simulink library "ConverterPlantLibrary"  (R2026a)
settings: Solver=VariableStepAuto
libraries: nesl_utility x213, fl_lib x211, ee_lib x205
(part 9 of 22)

== system ConverterPlantLibrary/Non-Isolated DC-DC Converters/Non-Isolated DC-DC Converter/NonIsolatedDCDCVariant/SynchronousBoost/MainSwitch/SwitchingMOSFETwithThermal ==
  G : Inport
  MOSFET : ee_lib/Semiconductors & Converters/MOSFET (Ideal, Switching)  PartSpecification="{\"CollectionId\":\"MW.SimscapeElectrical\",\"CollectionVersion\":\"1.0.0\",\"DatasetId\":\"Wolfspeed|C3M0010090K|\",\"DisplayName\":\"Wolfspeed:C3M0010090K\"}"  port_option=ee.enum.controlport.ps  Rds=0.03 % Datasheet derived Ohm  Goff=1e-05 S  Vth=2.4 % Wolfspeed XML derived V  diode_param=ee.enum.semiconductors.protectionDiode.nodynamics  diode_Vf=0.8 V  diode_Ron=1e-3 Ohm  diode_Goff=1e-5 S  diode_C=50e-9 % Parameter not set F  diode_iRM=-235 % Parameter not set A  diode_iF=300 % Parameter not set A  diode_idot=-50 % Parameter not set A/us  diode_trr_param=ee.enum.converters.diodeReverseParam.trr_factor  diode_trr_factor=3 % Parameter not set  diode_trr=15 % Parameter not set us  diode_Qrr=1500 % Parameter not set s*uA  ids_specify=off  ids_priority=None  ids=0 A  ids_nominal_specify=off  ids_nominal_value=1  ids_nominal_unit=A  vds_specify=off  vds_priority=None  vds=0 V  vds_nominal_specify=off  vds_nominal_value=1  vds_nominal_unit=V  vgs_specify=off  vgs_priority=None  vgs=0 V  vgs_nominal_specify=off  vgs_nominal_value=1  vgs_nominal_unit=V  thermal_loss_option=ee.enum.converters.thermalLossOption.tabulated2d  Von_data=[-2.582 -2.511 -2.366 -2.145 -1.916 -1.601 -1.356 -1.103 -0.7517 -0.4733 -0.3149 -0.1528 -0.0851 -0.05 0 0.094 0.161 0.305 0.51 0.83 1.31 1.61 1.908 2.42 2.766 3.142 3.373 3.713;-2.869 -2.757 -2.58 -2.311 -2.042 -1.683 -1.41 -1.134 -0.7615 -0.4747 -0.3153 -0.149 -0.0819 -0.0469 0 0.09975 0.154 0.303 0.509 0.819 1.241 1.581 1.9 2.39 2.758 3.144 3.4 3.78;-4.55 -4.355 -4.055 -3.569 -3.136 -2.526 -2.113 -1.659 -1.117 -0.7115 -0.4389 -0.2087 -0.116 -0.0674 0 0.123 0.239 0.421 0.701 1.175 1.743 2.252 2.7 3.4 4 4.52 5.03 5.4;-5.005 -4.791 -4.461 -3.926 -3.45 -2.779 -2.324 -1.825 -1.229 -0.7826 -0.4828 -0.2296 -0.1276 -0.07414 0 0.1353 0.2629 0.4631 0.7711 1.292 1.917 2.477 2.97 3.74 4.4 4.972 5.533 5.94] % Wolfspeed XML derived V  Tj=[-55 25 150 900] % Wolfspeed XML derived degC  Iout_data=[-311.6 -300 -280 -250 -220 -180 -150 -120 -80 -50 -32.71 -15.83 -9 -5.52 0 9 15.6 30 50 80 120 150 180 220 250 280 300 327] % Wolfspeed XML derived A  tabulateWithVds=true  Eon_data=[0 0.00054 0.00072 0.0009 0.00109 0.00126 0.00142 0.00163 0.0018;0 0.00036 0.00048 0.0006 0.00073 0.00084 0.00095 0.00109 0.0012;0 0.00037 0.00049 0.00061 0.00074 0.00085 0.00097 0.00111 0.00122;0 0.00041 0.00054 0.00067 0.00081 0.00094 0.00106 0.00122 0.00135;0 0.00041 0.00054 0.00067 0.00081 0.00094 0.00106 0.00122 0.00135] % Wolfspeed XML derived J  Eoff_data=[0 0.00013 0.0002 0.00022 0.00026 0.00033 0.00044 0.00055 0.00067;0 0.00014 0.00021 0.00024 0.00028 0.00036 0.00047 0.00059 0.00072;0 0.00016 0.00024 0.00027 0.00031 0.00041 0.00054 0.00067 0.00082;0 0.00016 0.00024 0.00027 0.00032 0.00041 0.00054 0.00068 0.00083;0 0.00016 0.00024 0.00027 0.00032 0.00041 0.00054 0.00068 0.00083] % Wolfspeed XML derived J  Eon_data_3D=reshape([0;0;0;0;0;0;0;0;0;0;0;0;0;0;0;0;0;0;0;0;0;0;0;0;0;0;0;0;0;0;0;0;0;0;0;0;0;0;0;0;0;0;0;0;0;0;0;0;0;0;0;0;0;0;0;0;0;0;0;0;0;0;0;0;0;0;0;0;0;0;0;0;0;0;0;0;0;0;0;0;0;0;0;0;0;0;0;0;0;0;0;0;0;0;0;0.00025;0.00017;0.00017;0.00019;0.00019;0.00035;0.00024;0.00024;0.00026;0.00026;0.00044;0.00029;0.0003;0.00033;0.00033;0.00051;0.00034;0.00035;0.00038;0.00038;0.0006;0.0004;0.00041;0.00045;0.00045;0.00072;0.00048;0.00049;0.00054;0.00054;0.00079;0.00053;0.00054;0.00059;0.00059;0.00087;0.00058;0.00059;0.00065;0.00065;0;0;0;0;0;0.00054;0.00036;0.00037;0.00041;0.00041;0.00072;0.00048;0.00049;0.00054;0.00054;0.0009;0.0006;0.00061;0.00067;0.00067;0.00109;0.00073;0.00074;0.00081;0.00081;0.00126;0.00084;0.00085;0.00094;0.00094;0.00142;0.00095;0.00097;0.00106;0.00106;0.00163;0.00109;0.00111;0.00122;0.00122;0.0018;0.0012;0.00122;0.00135;0.00135],[5 9 4]) % Wolfspeed XML derived J  Eoff_data_3D=reshape([0;0;0;0;0;0;0;0;0;0;0;0;0;0;0;0;0;0;0;0;0;0;0;0;0;0;0;0;0;0;0;0;0;0;0;0;0;0;0;0;0;0;0;0;0;0;0;0;0;0;0;0;0;0;0;0;0;0;0;0;0;0;0;0;0;0;0;0;0;0;0;0;0;0;0;0;0;0;0;0;0;0;0;0;0;0;0;0;0;0;0;0;0;0;0;8e-05;8e-05;0.0001;0.0001;0.0001;0.00014;0.00015;0.00017;0.00017;0.00017;0.00016;0.00018;0.0002;0.0002;0.0002;0.00017;0.00018;0.00021;0.00021;0.00021;0.00023;0.00025;0.00029;0.00029;0.00029;0.0003;0.00032;0.00037;0.00037;0.00037;0.00038;0.00041;0.00046;0.00047;0.00047;0.00046;0.00049;0.00056;0.00057;0.00057;0;0;0;0;0;0.00013;0.00014;0.00016;0.00016;0.00016;0.0002;0.00021;0.00024;0.00024;0.00024;0.00022;0.00024;0.00027;0.00027;0.00027;0.00026;0.00028;0.00031;0.00032;0.00032;0.00033;0.00036;0.00041;0.00041;0.00041;0.00044;0.00047;0.00054;0.00054;0.00054;0.00055;0.00059;0.00067;0.00068;0.00068;0.00067;0.00072;0.00082;0.00083;0.00083],[5 9 4]) % Wolfspeed XML derived J  Tj_loss=[-55 25 150 900 1000] % Wolfspeed XML derived degC  Iout_data_loss=[0 12.2 26.4 38.8 52.6 66 78.9 91 103.3] % Wolfspeed XML derived A  Vds_loss=[-100 0 400 600] % Wolfspeed XML derived V  Eon_scalar=22.86e-3 % Parameter not set J  Eoff_scalar=17.14e-3 % Parameter not set J  Voff=300 % Parameter not set V  Iout_scalar=600 % Parameter not set A  useCurrentFromPreviousCycle=false % Parameter not set  useVoltageFromPreviousCycle=false % Parameter not set  diodeModelType=ee.enum.converters.diodeModelType.pwl  diodeTableType=ee.enum.diode.tableType.VfMat  diode_ReverseIVType=ee.enum.diode.diodeReverseIV.constant  diode_IfMat=[.07, .12, .19, 1.75, 4.24, 7.32, 11.2; .16, .3, .72, 2.14, 4.02, 6.35, 9.12] % Parameter not set A  diode_VfMat=[0 0.718 3.358 3.487 3.935 4.083 4.682 5.031 5.458 5.658 5.958 6.147 6.32 6.575 6.799 7.03 7.267 7.29;0 0.718 2.914 3.116 3.391 3.497 3.954 4.289 4.612 4.933 5.187 5.39 5.581 5.763 6.107 6.422 6.711 6.76;0 0.718 2.4 2.6 2.8 2.982 3.45 3.789 4.099 4.428 4.661 4.85 5.035 5.233 5.51 5.855 6.14 6.19;0 0.6462 2.16 2.34 2.52 2.684 3.105 3.41 3.689 3.985 4.195 4.365 4.532 4.71 4.959 5.269 5.526 5.571;0 0.6462 2.16 2.34 2.52 2.684 3.105 3.41 3.689 3.985 4.195 4.365 4.532 4.71 4.959 5.269 5.526 5.571] % Wolfspeed XML derived V  diode_TjVec=[-55 25 150 900 1000] % Wolfspeed XML derived degC  diode_VfVec=[.5, .7, .9, 1.3, 1.7, 2.1, 2.5] % Parameter not set V  diode_IfVec=[0 0.21 1.74 3.58 8.82 11.74 29.79 49.06 71.98 98.06 121.2 141.4 161.2 181.3 221.3 260.9 300 306.3] % Wolfspeed XML derived A  diode_IrMat=[1e-06, 2e-06, 5e-06, 1e-05, 2.5e-05, 5e-05, .0001; 2e-06, 5e-06, 1e-05, 4e-05, 8e-05, .0002, .0005] % Parameter not set A  diode_VrMat=[10, 100, 200, 250, 300, 325, 350; 10, 70, 160, 220, 270, 300, 320] % Parameter not set V  diode_VrVec=[10, 20, 40, 50, 70, 80, 100] % Parameter not set V  diode_IrVec=[1e-06, 2e-06, 5e-06, 1e-05, 2e-05, 5e-05, .0001] % Parameter not set A  diode_Vr=-600 % Parameter not set V  diode_Ls=150 % Parameter not set nH  diode_Erec=0.03 % Parameter not set J  diode_rec_loss_model=ee.enum.diode.reverseRecoveryModel.fixed  diode_ErecVal=0 % Parameter not set J  diode_scaleWithIandV=false  diode_ErecMat=[0 0;0 0] % Wolfspeed XML derived J  diodeErecMat3D=zeros(2, 3, 2) J  diode_TjrecVec=[25 35] % Wolfspeed XML derived degC  diode_IfrecVec=[0 10] % Wolfspeed XML derived A  diodeVrecVec=[0, 100] V  diode_IrecVal=10 % Parameter not set A  diode_VrecVal=10 % Wolfspeed XML derived V  diode_tFilter=1 / 1000 / 100 % Parameter not set s  separateThermalPortForDiode=false  thermal_network_parameterization=ee.enum.thermalNetworkTopology.external  Rth=[.03, .2] % Parameter not set K/W  Rth_Cauer=[0.01728 0.0646 0.05315 0.1045] % Wolfspeed XML derived K/W  Rth_Foster=[.08, .14, .22, .16] % Parameter not set K/W  thermal_mass_parameterization=ee.enum.thermalNetwork.thermalmass  thermal_mass=[3, 25] % Parameter not set J/K  thermal_mass_Cauer=[0.00466 0.0158 0.0642 0.264] % Wolfspeed XML derived J/K  thermal_mass_Foster=[.001, .005, .05, .5] % Parameter not set J/K  thermal_time_constant=[.1, 5] % Parameter not set s  thermal_time_constant_Cauer=[.1, 1, 5] % Parameter not set s  thermal_time_constant_Foster=[7e-05, .0007, .01, .08] % Parameter not set s  thermal_mass_initial_temperatures=[25, 25] % Parameter not set degC  thermal_mass_initial_temperatures_Cauer=[25 25 25 25] % Wolfspeed XML derived degC  junction_thermal_mass=0.01 % Parameter not set J/K  Tvec_initial_Foster=[25, 25, 25, 25] % Parameter not set degC  RthDiode=[.03, .2] % Parameter not set K/W  RthCauerDiode=[0.01728 0.0646 0.05315 0.1045] % Wolfspeed XML derived K/W  RthFosterDiode=[.03, .2] % Parameter not set K/W  thermalMassDiode=[3, 25] % Parameter not set J/K  thermalMassCauerDiode=[0.00466 0.0158 0.0642 0.264] % Wolfspeed XML derived J/K  thermalMassFosterDiode=[33, 50] % Parameter not set J/K  thermalTauDiode=[.1, 5] % Parameter not set s  thermalTauCauerDiode=[.1, 1, 5] % Parameter not set s  thermalTauFosterDiode=[1, 10] % Parameter not set s  thermalMassInitTempDiode=[25, 25] % Parameter not set degC  thermalMassInitTempCauerDiode=[25 25 25 25] % Wolfspeed XML derived degC  junctionthermalMassDiode=0.1 % Parameter not set J/K  TVecInitialFosterDiode=[25, 25, 25, 25] % Parameter not set degC  no_thermal_network=0 % Parameter not set  mosfet_junction_temperature_specify=on  mosfet_junction_temperature_priority=High  mosfet_junction_temperature=simTemp_K K  mosfet_junction_temperature_nominal_specify=off  mosfet_junction_temperature_nominal_value=1  mosfet_junction_temperature_nominal_unit=degC  diode_junction_temperature_specify=off  diode_junction_temperature_priority=None  diode_junction_temperature=simTemp_K K  diode_junction_temperature_nominal_specify=off  diode_junction_temperature_nominal_value=1  diode_junction_temperature_nominal_unit=degC  Qj_specify=off  Qj_priority=None  Qj=0 W  Qj_nominal_specify=off  Qj_nominal_value=1  Qj_nominal_unit=W  accumulatedSwitchingLosses_specify=off  accumulatedSwitchingLosses_priority=None  accumulatedSwitchingLosses=0 J
      settings: AttributesFormatString=Wolfspeed:C3M0010090K
  SL_PS : nesl_utility/Simulink-PS Converter  PhysicalDomain=network_engine_domain  SubClassName=ps_input  LeftPortType=input  RightPortType=output  PseudoPeriodic=off  Frequencies=[]  NoiseDistribution=none  NoiseParameters=[]  Unit=1  AffineConversion=off  FilteringAndDerivatives=provide  SimscapeFilterOrder=1  InputFilterTimeConstant=0.001  UdotUserProvided=0
  Temperature Source : fl_lib/Thermal/Thermal Sources/Temperature Source  temperature=simTemp_K K
  Thermal Resistor : ee_lib/Passive/Thermal/Thermal Resistor  R=1e-3 K/W  T_specify=off  T_priority=None  T=0 K  T_nominal_specify=off  T_nominal_value=1  T_nominal_unit=K  Q_specify=off  Q_priority=None  Q=0 W  Q_nominal_specify=off  Q_nominal_value=1  Q_nominal_unit=W
  D : PMIOPort  Side=Left
  S : PMIOPort  Port=2  Side=Right
  wires:
  G/1 -> SL_PS/1
  connections:
  Thermal Resistor/RConn1 -- Temperature Source/LConn1
  MOSFET/LConn2 -- Thermal Resistor/LConn1
  MOSFET/RConn2 -- S/RConn1
  MOSFET/RConn1 -- D/RConn1
  SL_PS/RConn1 -- MOSFET/LConn1

== system ConverterPlantLibrary/Non-Isolated DC-DC Converters/Non-Isolated DC-DC Converter/NonIsolatedDCDCVariant/SynchronousBoost/SyncSwitch/IdealSwitch ==
  G : Inport
  SL_PS : nesl_utility/Simulink-PS Converter  PhysicalDomain=network_engine_domain  SubClassName=ps_input  LeftPortType=input  RightPortType=output  PseudoPeriodic=off  Frequencies=[]  NoiseDistribution=none  NoiseParameters=[]  Unit=1  AffineConversion=off  FilteringAndDerivatives=provide  SimscapeFilterOrder=1  InputFilterTimeConstant=0.001  UdotUserProvided=0
  Switch : ee_lib/Semiconductors & Converters/Ideal Semiconductor Switch  port_option=ee.enum.controlport.ps  Ron=RdsOn_SI Ohm  Goff=GdsOff_SI 1/Ohm  Vth=Vth_SI V  diode_param=ee.enum.semiconductors.protectionDiode.nodynamics  diode_Vf=VfBody_SI V  diode_Ron=RdBody_SI Ohm  diode_Goff=GdBody_SI 1/Ohm  diode_C=50e-9 F  diode_iRM=-235 A  diode_iF=300 A  diode_idot=-50 A/us  diode_trr_param=ee.enum.converters.diodetrr.trr_factor  diode_trr_factor=3  diode_trr=15 us  diode_Qrr=1500 s*uA
  D : PMIOPort  Side=Left
  S : PMIOPort  Port=2  Side=Right
  wires:
  G/1 -> SL_PS/1
  connections:
  Switch/RConn2 -- S/RConn1
  Switch/RConn1 -- D/RConn1
  SL_PS/RConn1 -- Switch/LConn1

== system ConverterPlantLibrary/Non-Isolated DC-DC Converters/Non-Isolated DC-DC Converter/NonIsolatedDCDCVariant/SynchronousBoost/SyncSwitch/SwitchingMOSFETwithThermal ==
  G : Inport
  MOSFET : ee_lib/Semiconductors & Converters/MOSFET (Ideal, Switching)  PartSpecification="{\"CollectionId\":\"SimscapeElectrical\",\"CollectionVersion\":\"1.0.0\",\"DatasetId\":\"Wolfspeed|C3M0010090K|\",\"DisplayName\":\"Wolfspeed:C3M0010090K\"}"  port_option=ee.enum.controlport.ps  Rds=0.03 % Datasheet derived Ohm  Goff=1e-05 S  Vth=2.4 % Wolfspeed XML derived V  diode_param=ee.enum.semiconductors.protectionDiode.nodynamics  diode_Vf=0.8 V  diode_Ron=1e-3 Ohm  diode_Goff=1e-5 S  diode_C=50e-9 % Parameter not set F  diode_iRM=-235 % Parameter not set A  diode_iF=300 % Parameter not set A  diode_idot=-50 % Parameter not set A/us  diode_trr_param=ee.enum.converters.diodeReverseParam.trr_factor  diode_trr_factor=3 % Parameter not set  diode_trr=15 % Parameter not set us  diode_Qrr=1500 % Parameter not set s*uA  ids_specify=off  ids_priority=None  ids=0 A  ids_nominal_specify=off  ids_nominal_value=1  ids_nominal_unit=A  vds_specify=off  vds_priority=None  vds=0 V  vds_nominal_specify=off  vds_nominal_value=1  vds_nominal_unit=V  vgs_specify=off  vgs_priority=None  vgs=0 V  vgs_nominal_specify=off  vgs_nominal_value=1  vgs_nominal_unit=V  thermal_loss_option=ee.enum.converters.thermalLossOption.tabulated2d  Von_data=[-2.582 -2.511 -2.366 -2.145 -1.916 -1.601 -1.356 -1.103 -0.7517 -0.4733 -0.3149 -0.1528 -0.0851 -0.05 0 0.094 0.161 0.305 0.51 0.83 1.31 1.61 1.908 2.42 2.766 3.142 3.373 3.713;-2.869 -2.757 -2.58 -2.311 -2.042 -1.683 -1.41 -1.134 -0.7615 -0.4747 -0.3153 -0.149 -0.0819 -0.0469 0 0.09975 0.154 0.303 0.509 0.819 1.241 1.581 1.9 2.39 2.758 3.144 3.4 3.78;-4.55 -4.355 -4.055 -3.569 -3.136 -2.526 -2.113 -1.659 -1.117 -0.7115 -0.4389 -0.2087 -0.116 -0.0674 0 0.123 0.239 0.421 0.701 1.175 1.743 2.252 2.7 3.4 4 4.52 5.03 5.4;-5.005 -4.791 -4.461 -3.926 -3.45 -2.779 -2.324 -1.825 -1.229 -0.7826 -0.4828 -0.2296 -0.1276 -0.07414 0 0.1353 0.2629 0.4631 0.7711 1.292 1.917 2.477 2.97 3.74 4.4 4.972 5.533 5.94] % Wolfspeed XML derived V  Tj=[-55 25 150 900] % Wolfspeed XML derived degC  Iout_data=[-311.6 -300 -280 -250 -220 -180 -150 -120 -80 -50 -32.71 -15.83 -9 -5.52 0 9 15.6 30 50 80 120 150 180 220 250 280 300 327] % Wolfspeed XML derived A  tabulateWithVds=true  Eon_data=[0 0.00054 0.00072 0.0009 0.00109 0.00126 0.00142 0.00163 0.0018;0 0.00036 0.00048 0.0006 0.00073 0.00084 0.00095 0.00109 0.0012;0 0.00037 0.00049 0.00061 0.00074 0.00085 0.00097 0.00111 0.00122;0 0.00041 0.00054 0.00067 0.00081 0.00094 0.00106 0.00122 0.00135;0 0.00041 0.00054 0.00067 0.00081 0.00094 0.00106 0.00122 0.00135] % Wolfspeed XML derived J  Eoff_data=[0 0.00013 0.0002 0.00022 0.00026 0.00033 0.00044 0.00055 0.00067;0 0.00014 0.00021 0.00024 0.00028 0.00036 0.00047 0.00059 0.00072;0 0.00016 0.00024 0.00027 0.00031 0.00041 0.00054 0.00067 0.00082;0 0.00016 0.00024 0.00027 0.00032 0.00041 0.00054 0.00068 0.00083;0 0.00016 0.00024 0.00027 0.00032 0.00041 0.00054 0.00068 0.00083] % Wolfspeed XML derived J  Eon_data_3D=reshape([0;0;0;0;0;0;0;0;0;0;0;0;0;0;0;0;0;0;0;0;0;0;0;0;0;0;0;0;0;0;0;0;0;0;0;0;0;0;0;0;0;0;0;0;0;0;0;0;0;0;0;0;0;0;0;0;0;0;0;0;0;0;0;0;0;0;0;0;0;0;0;0;0;0;0;0;0;0;0;0;0;0;0;0;0;0;0;0;0;0;0;0;0;0;0;0.00025;0.00017;0.00017;0.00019;0.00019;0.00035;0.00024;0.00024;0.00026;0.00026;0.00044;0.00029;0.0003;0.00033;0.00033;0.00051;0.00034;0.00035;0.00038;0.00038;0.0006;0.0004;0.00041;0.00045;0.00045;0.00072;0.00048;0.00049;0.00054;0.00054;0.00079;0.00053;0.00054;0.00059;0.00059;0.00087;0.00058;0.00059;0.00065;0.00065;0;0;0;0;0;0.00054;0.00036;0.00037;0.00041;0.00041;0.00072;0.00048;0.00049;0.00054;0.00054;0.0009;0.0006;0.00061;0.00067;0.00067;0.00109;0.00073;0.00074;0.00081;0.00081;0.00126;0.00084;0.00085;0.00094;0.00094;0.00142;0.00095;0.00097;0.00106;0.00106;0.00163;0.00109;0.00111;0.00122;0.00122;0.0018;0.0012;0.00122;0.00135;0.00135],[5 9 4]) % Wolfspeed XML derived J  Eoff_data_3D=reshape([0;0;0;0;0;0;0;0;0;0;0;0;0;0;0;0;0;0;0;0;0;0;0;0;0;0;0;0;0;0;0;0;0;0;0;0;0;0;0;0;0;0;0;0;0;0;0;0;0;0;0;0;0;0;0;0;0;0;0;0;0;0;0;0;0;0;0;0;0;0;0;0;0;0;0;0;0;0;0;0;0;0;0;0;0;0;0;0;0;0;0;0;0;0;0;8e-05;8e-05;0.0001;0.0001;0.0001;0.00014;0.00015;0.00017;0.00017;0.00017;0.00016;0.00018;0.0002;0.0002;0.0002;0.00017;0.00018;0.00021;0.00021;0.00021;0.00023;0.00025;0.00029;0.00029;0.00029;0.0003;0.00032;0.00037;0.00037;0.00037;0.00038;0.00041;0.00046;0.00047;0.00047;0.00046;0.00049;0.00056;0.00057;0.00057;0;0;0;0;0;0.00013;0.00014;0.00016;0.00016;0.00016;0.0002;0.00021;0.00024;0.00024;0.00024;0.00022;0.00024;0.00027;0.00027;0.00027;0.00026;0.00028;0.00031;0.00032;0.00032;0.00033;0.00036;0.00041;0.00041;0.00041;0.00044;0.00047;0.00054;0.00054;0.00054;0.00055;0.00059;0.00067;0.00068;0.00068;0.00067;0.00072;0.00082;0.00083;0.00083],[5 9 4]) % Wolfspeed XML derived J  Tj_loss=[-55 25 150 900 1000] % Wolfspeed XML derived degC  Iout_data_loss=[0 12.2 26.4 38.8 52.6 66 78.9 91 103.3] % Wolfspeed XML derived A  Vds_loss=[-100 0 400 600] % Wolfspeed XML derived V  Eon_scalar=22.86e-3 % Parameter not set J  Eoff_scalar=17.14e-3 % Parameter not set J  Voff=300 % Parameter not set V  Iout_scalar=600 % Parameter not set A  useCurrentFromPreviousCycle=false % Parameter not set  useVoltageFromPreviousCycle=false % Parameter not set  diodeModelType=ee.enum.converters.diodeModelType.pwl  diodeTableType=ee.enum.diode.tableType.VfMat  diode_ReverseIVType=ee.enum.diode.diodeReverseIV.constant  diode_IfMat=[.07, .12, .19, 1.75, 4.24, 7.32, 11.2; .16, .3, .72, 2.14, 4.02, 6.35, 9.12] % Parameter not set A  diode_VfMat=[0 0.718 3.358 3.487 3.935 4.083 4.682 5.031 5.458 5.658 5.958 6.147 6.32 6.575 6.799 7.03 7.267 7.29;0 0.718 2.914 3.116 3.391 3.497 3.954 4.289 4.612 4.933 5.187 5.39 5.581 5.763 6.107 6.422 6.711 6.76;0 0.718 2.4 2.6 2.8 2.982 3.45 3.789 4.099 4.428 4.661 4.85 5.035 5.233 5.51 5.855 6.14 6.19;0 0.6462 2.16 2.34 2.52 2.684 3.105 3.41 3.689 3.985 4.195 4.365 4.532 4.71 4.959 5.269 5.526 5.571;0 0.6462 2.16 2.34 2.52 2.684 3.105 3.41 3.689 3.985 4.195 4.365 4.532 4.71 4.959 5.269 5.526 5.571] % Wolfspeed XML derived V  diode_TjVec=[-55 25 150 900 1000] % Wolfspeed XML derived degC  diode_VfVec=[.5, .7, .9, 1.3, 1.7, 2.1, 2.5] % Parameter not set V  diode_IfVec=[0 0.21 1.74 3.58 8.82 11.74 29.79 49.06 71.98 98.06 121.2 141.4 161.2 181.3 221.3 260.9 300 306.3] % Wolfspeed XML derived A  diode_IrMat=[1e-06, 2e-06, 5e-06, 1e-05, 2.5e-05, 5e-05, .0001; 2e-06, 5e-06, 1e-05, 4e-05, 8e-05, .0002, .0005] % Parameter not set A  diode_VrMat=[10, 100, 200, 250, 300, 325, 350; 10, 70, 160, 220, 270, 300, 320] % Parameter not set V  diode_VrVec=[10, 20, 40, 50, 70, 80, 100] % Parameter not set V  diode_IrVec=[1e-06, 2e-06, 5e-06, 1e-05, 2e-05, 5e-05, .0001] % Parameter not set A  diode_Vr=-600 % Parameter not set V  diode_Ls=150 % Parameter not set nH  diode_Erec=0.03 % Parameter not set J  diode_rec_loss_model=ee.enum.diode.reverseRecoveryModel.fixed  diode_ErecVal=0 % Parameter not set J  diode_scaleWithIandV=false  diode_ErecMat=[0 0;0 0] % Wolfspeed XML derived J  diodeErecMat3D=zeros(2, 3, 2) J  diode_TjrecVec=[25 35] % Wolfspeed XML derived degC  diode_IfrecVec=[0 10] % Wolfspeed XML derived A  diodeVrecVec=[0, 100] V  diode_IrecVal=10 % Parameter not set A  diode_VrecVal=10 % Wolfspeed XML derived V  diode_tFilter=1 / 1000 / 100 % Parameter not set s  separateThermalPortForDiode=false  thermal_network_parameterization=ee.enum.thermalNetworkTopology.external  Rth=[.03, .2] % Parameter not set K/W  Rth_Cauer=[0.01728 0.0646 0.05315 0.1045] % Wolfspeed XML derived K/W  Rth_Foster=[.08, .14, .22, .16] % Parameter not set K/W  thermal_mass_parameterization=ee.enum.thermalNetwork.thermalmass  thermal_mass=[3, 25] % Parameter not set J/K  thermal_mass_Cauer=[0.00466 0.0158 0.0642 0.264] % Wolfspeed XML derived J/K  thermal_mass_Foster=[.001, .005, .05, .5] % Parameter not set J/K  thermal_time_constant=[.1, 5] % Parameter not set s  thermal_time_constant_Cauer=[.1, 1, 5] % Parameter not set s  thermal_time_constant_Foster=[7e-05, .0007, .01, .08] % Parameter not set s  thermal_mass_initial_temperatures=[25, 25] % Parameter not set degC  thermal_mass_initial_temperatures_Cauer=[25 25 25 25] % Wolfspeed XML derived degC  junction_thermal_mass=0.01 % Parameter not set J/K  Tvec_initial_Foster=[25, 25, 25, 25] % Parameter not set degC  RthDiode=[.03, .2] % Parameter not set K/W  RthCauerDiode=[0.01728 0.0646 0.05315 0.1045] % Wolfspeed XML derived K/W  RthFosterDiode=[.03, .2] % Parameter not set K/W  thermalMassDiode=[3, 25] % Parameter not set J/K  thermalMassCauerDiode=[0.00466 0.0158 0.0642 0.264] % Wolfspeed XML derived J/K  thermalMassFosterDiode=[33, 50] % Parameter not set J/K  thermalTauDiode=[.1, 5] % Parameter not set s  thermalTauCauerDiode=[.1, 1, 5] % Parameter not set s  thermalTauFosterDiode=[1, 10] % Parameter not set s  thermalMassInitTempDiode=[25, 25] % Parameter not set degC  thermalMassInitTempCauerDiode=[25 25 25 25] % Wolfspeed XML derived degC  junctionthermalMassDiode=0.1 % Parameter not set J/K  TVecInitialFosterDiode=[25, 25, 25, 25] % Parameter not set degC  no_thermal_network=0 % Parameter not set  mosfet_junction_temperature_specify=on  mosfet_junction_temperature_priority=High  mosfet_junction_temperature=simTemp_K K  mosfet_junction_temperature_nominal_specify=off  mosfet_junction_temperature_nominal_value=1  mosfet_junction_temperature_nominal_unit=degC  diode_junction_temperature_specify=off  diode_junction_temperature_priority=None  diode_junction_temperature=simTemp_K K  diode_junction_temperature_nominal_specify=off  diode_junction_temperature_nominal_value=1  diode_junction_temperature_nominal_unit=degC  Qj_specify=off  Qj_priority=None  Qj=0 W  Qj_nominal_specify=off  Qj_nominal_value=1  Qj_nominal_unit=W  accumulatedSwitchingLosses_specify=off  accumulatedSwitchingLosses_priority=None  accumulatedSwitchingLosses=0 J
      settings: AttributesFormatString=Wolfspeed:C3M0010090K
  SL_PS : nesl_utility/Simulink-PS Converter  PhysicalDomain=network_engine_domain  SubClassName=ps_input  LeftPortType=input  RightPortType=output  PseudoPeriodic=off  Frequencies=[]  NoiseDistribution=none  NoiseParameters=[]  Unit=1  AffineConversion=off  FilteringAndDerivatives=provide  SimscapeFilterOrder=1  InputFilterTimeConstant=0.001  UdotUserProvided=0
  Temperature Source : fl_lib/Thermal/Thermal Sources/Temperature Source  temperature=simTemp_K K
  Thermal Resistor : ee_lib/Passive/Thermal/Thermal Resistor  R=1e-3 K/W  T_specify=off  T_priority=None  T=0 K  T_nominal_specify=off  T_nominal_value=1  T_nominal_unit=K  Q_specify=off  Q_priority=None  Q=0 W  Q_nominal_specify=off  Q_nominal_value=1  Q_nominal_unit=W
  D : PMIOPort  Side=Left
  S : PMIOPort  Port=2  Side=Right
  wires:
  G/1 -> SL_PS/1
  connections:
  Thermal Resistor/RConn1 -- Temperature Source/LConn1
  MOSFET/LConn2 -- Thermal Resistor/LConn1
  MOSFET/RConn2 -- S/RConn1
  MOSFET/RConn1 -- D/RConn1
  SL_PS/RConn1 -- MOSFET/LConn1

== system ConverterPlantLibrary/Non-Isolated DC-DC Converters/Non-Isolated DC-DC Converter/NonIsolatedDCDCVariant/SynchronousBuck/MainSwitch/IdealSwitch ==
  G : Inport
  SL_PS : nesl_utility/Simulink-PS Converter  PhysicalDomain=network_engine_domain  SubClassName=ps_input  LeftPortType=input  RightPortType=output  PseudoPeriodic=off  Frequencies=[]  NoiseDistribution=none  NoiseParameters=[]  Unit=1  AffineConversion=off  FilteringAndDerivatives=provide  SimscapeFilterOrder=1  InputFilterTimeConstant=0.001  UdotUserProvided=0
  Switch : ee_lib/Semiconductors & Converters/Ideal Semiconductor Switch  port_option=ee.enum.controlport.ps  Ron=RdsOn_SI Ohm  Goff=GdsOff_SI 1/Ohm  Vth=Vth_SI V  diode_param=ee.enum.semiconductors.protectionDiode.nodynamics  diode_Vf=VfBody_SI V  diode_Ron=RdBody_SI Ohm  diode_Goff=GdBody_SI 1/Ohm  diode_C=50e-9 F  diode_iRM=-235 A  diode_iF=300 A  diode_idot=-50 A/us  diode_trr_param=ee.enum.converters.diodetrr.trr_factor  diode_trr_factor=3  diode_trr=15 us  diode_Qrr=1500 s*uA
  D : PMIOPort  Side=Left
  S : PMIOPort  Port=2  Side=Right
  wires:
  G/1 -> SL_PS/1
  connections:
  SL_PS/RConn1 -- Switch/LConn1
  Switch/RConn1 -- D/RConn1
  Switch/RConn2 -- S/RConn1

== system ConverterPlantLibrary/Non-Isolated DC-DC Converters/Non-Isolated DC-DC Converter/NonIsolatedDCDCVariant/SynchronousBuck/MainSwitch/SwitchingMOSFETwithThermal ==
  G : Inport
  MOSFET : ee_lib/Semiconductors & Converters/MOSFET (Ideal, Switching)  PartSpecification="{\"CollectionId\":\"MW.SimscapeElectrical\",\"CollectionVersion\":\"1.0.0\",\"DatasetId\":\"Wolfspeed|C3M0010090K|\",\"DisplayName\":\"Wolfspeed:C3M0010090K\"}"  port_option=ee.enum.controlport.ps  Rds=0.03 % Datasheet derived Ohm  Goff=1e-05 S  Vth=2.41 % Wolfspeed XML derived V  diode_param=ee.enum.semiconductors.protectionDiode.nodynamics  diode_Vf=0.8 V  diode_Ron=1e-3 Ohm  diode_Goff=1e-5 S  diode_C=50e-9 % Parameter not set F  diode_iRM=-235 % Parameter not set A  diode_iF=300 % Parameter not set A  diode_idot=-50 % Parameter not set A/us  diode_trr_param=ee.enum.converters.diodeReverseParam.trr_factor  diode_trr_factor=3 % Parameter not set  diode_trr=15 % Parameter not set us  diode_Qrr=1500 % Parameter not set s*uA  ids_specify=off  ids_priority=None  ids=0 A  ids_nominal_specify=off  ids_nominal_value=1  ids_nominal_unit=A  vds_specify=off  vds_priority=None  vds=0 V  vds_nominal_specify=off  vds_nominal_value=1  vds_nominal_unit=V  vgs_specify=off  vgs_priority=None  vgs=0 V  vgs_nominal_specify=off  vgs_nominal_value=1  vgs_nominal_unit=V  thermal_loss_option=ee.enum.converters.thermalLossOption.tabulated2d  Von_data=[-2.582 -2.511 -2.366 -2.145 -1.916 -1.601 -1.356 -1.103 -0.7517 -0.4733 -0.3149 -0.1528 -0.0851 -0.05 0 0.094 0.161 0.305 0.51 0.83 1.31 1.61 1.908 2.42 2.766 3.142 3.373 3.713;-2.869 -2.757 -2.58 -2.311 -2.042 -1.683 -1.41 -1.134 -0.7615 -0.4747 -0.3153 -0.149 -0.0819 -0.0469 0 0.09975 0.154 0.303 0.509 0.819 1.241 1.581 1.9 2.39 2.758 3.144 3.4 3.78;-4.55 -4.355 -4.055 -3.569 -3.136 -2.526 -2.113 -1.659 -1.117 -0.7115 -0.4389 -0.2087 -0.116 -0.0674 0 0.123 0.239 0.421 0.701 1.175 1.743 2.252 2.7 3.4 4 4.52 5.03 5.4;-5.005 -4.791 -4.461 -3.926 -3.45 -2.779 -2.324 -1.825 -1.229 -0.7826 -0.4828 -0.2296 -0.1276 -0.07414 0 0.1353 0.2629 0.4631 0.7711 1.292 1.917 2.477 2.97 3.74 4.4 4.972 5.533 5.94] % Wolfspeed XML derived V  Tj=[-55 25 150 900] % Wolfspeed XML derived degC  Iout_data=[-311.6 -300 -280 -250 -220 -180 -150 -120 -80 -50 -32.71 -15.83 -9 -5.52 0 9 15.6 30 50 80 120 150 180 220 250 280 300 327] % Wolfspeed XML derived A  tabulateWithVds=true  Eon_data=[0 0.00054 0.00072 0.0009 0.00109 0.00126 0.00142 0.00163 0.0018;0 0.00036 0.00048 0.0006 0.00073 0.00084 0.00095 0.00109 0.0012;0 0.00037 0.00049 0.00061 0.00074 0.00085 0.00097 0.00111 0.00122;0 0.00041 0.00054 0.00067 0.00081 0.00094 0.00106 0.00122 0.00135;0 0.00041 0.00054 0.00067 0.00081 0.00094 0.00106 0.00122 0.00135] % Wolfspeed XML derived J  Eoff_data=[0 0.00013 0.0002 0.00022 0.00026 0.00033 0.00044 0.00055 0.00067;0 0.00014 0.00021 0.00024 0.00028 0.00036 0.00047 0.00059 0.00072;0 0.00016 0.00024 0.00027 0.00031 0.00041 0.00054 0.00067 0.00082;0 0.00016 0.00024 0.00027 0.00032 0.00041 0.00054 0.00068 0.00083;0 0.00016 0.00024 0.00027 0.00032 0.00041 0.00054 0.00068 0.00083] % Wolfspeed XML derived J  Eon_data_3D=reshape([0;0;0;0;0;0;0;0;0;0;0;0;0;0;0;0;0;0;0;0;0;0;0;0;0;0;0;0;0;0;0;0;0;0;0;0;0;0;0;0;0;0;0;0;0;0;0;0;0;0;0;0;0;0;0;0;0;0;0;0;0;0;0;0;0;0;0;0;0;0;0;0;0;0;0;0;0;0;0;0;0;0;0;0;0;0;0;0;0;0;0;0;0;0;0;0.00025;0.00017;0.00017;0.00019;0.00019;0.00035;0.00024;0.00024;0.00026;0.00026;0.00044;0.00029;0.0003;0.00033;0.00033;0.00051;0.00034;0.00035;0.00038;0.00038;0.0006;0.0004;0.00041;0.00045;0.00045;0.00072;0.00048;0.00049;0.00054;0.00054;0.00079;0.00053;0.00054;0.00059;0.00059;0.00087;0.00058;0.00059;0.00065;0.00065;0;0;0;0;0;0.00054;0.00036;0.00037;0.00041;0.00041;0.00072;0.00048;0.00049;0.00054;0.00054;0.0009;0.0006;0.00061;0.00067;0.00067;0.00109;0.00073;0.00074;0.00081;0.00081;0.00126;0.00084;0.00085;0.00094;0.00094;0.00142;0.00095;0.00097;0.00106;0.00106;0.00163;0.00109;0.00111;0.00122;0.00122;0.0018;0.0012;0.00122;0.00135;0.00135],[5 9 4]) % Wolfspeed XML derived J  Eoff_data_3D=reshape([0;0;0;0;0;0;0;0;0;0;0;0;0;0;0;0;0;0;0;0;0;0;0;0;0;0;0;0;0;0;0;0;0;0;0;0;0;0;0;0;0;0;0;0;0;0;0;0;0;0;0;0;0;0;0;0;0;0;0;0;0;0;0;0;0;0;0;0;0;0;0;0;0;0;0;0;0;0;0;0;0;0;0;0;0;0;0;0;0;0;0;0;0;0;0;8e-05;8e-05;0.0001;0.0001;0.0001;0.00014;0.00015;0.00017;0.00017;0.00017;0.00016;0.00018;0.0002;0.0002;0.0002;0.00017;0.00018;0.00021;0.00021;0.00021;0.00023;0.00025;0.00029;0.00029;0.00029;0.0003;0.00032;0.00037;0.00037;0.00037;0.00038;0.00041;0.00046;0.00047;0.00047;0.00046;0.00049;0.00056;0.00057;0.00057;0;0;0;0;0;0.00013;0.00014;0.00016;0.00016;0.00016;0.0002;0.00021;0.00024;0.00024;0.00024;0.00022;0.00024;0.00027;0.00027;0.00027;0.00026;0.00028;0.00031;0.00032;0.00032;0.00033;0.00036;0.00041;0.00041;0.00041;0.00044;0.00047;0.00054;0.00054;0.00054;0.00055;0.00059;0.00067;0.00068;0.00068;0.00067;0.00072;0.00082;0.00083;0.00083],[5 9 4]) % Wolfspeed XML derived J  Tj_loss=[-55 25 150 900 1000] % Wolfspeed XML derived degC  Iout_data_loss=[0 12.2 26.4 38.8 52.6 66 78.9 91 103.3] % Wolfspeed XML derived A  Vds_loss=[-100 0 400 600] % Wolfspeed XML derived V  Eon_scalar=22.86e-3 % Parameter not set J  Eoff_scalar=17.14e-3 % Parameter not set J  Voff=300 % Parameter not set V  Iout_scalar=600 % Parameter not set A  useCurrentFromPreviousCycle=false % Parameter not set  useVoltageFromPreviousCycle=false % Parameter not set  diodeModelType=ee.enum.converters.diodeModelType.pwl  diodeTableType=ee.enum.diode.tableType.VfMat  diode_ReverseIVType=ee.enum.diode.diodeReverseIV.constant  diode_IfMat=[.07, .12, .19, 1.75, 4.24, 7.32, 11.2; .16, .3, .72, 2.14, 4.02, 6.35, 9.12] % Parameter not set A  diode_VfMat=[0 0.718 3.358 3.487 3.935 4.083 4.682 5.031 5.458 5.658 5.958 6.147 6.32 6.575 6.799 7.03 7.267 7.29;0 0.718 2.914 3.116 3.391 3.497 3.954 4.289 4.612 4.933 5.187 5.39 5.581 5.763 6.107 6.422 6.711 6.76;0 0.718 2.4 2.6 2.8 2.982 3.45 3.789 4.099 4.428 4.661 4.85 5.035 5.233 5.51 5.855 6.14 6.19;0 0.6462 2.16 2.34 2.52 2.684 3.105 3.41 3.689 3.985 4.195 4.365 4.532 4.71 4.959 5.269 5.526 5.571;0 0.6462 2.16 2.34 2.52 2.684 3.105 3.41 3.689 3.985 4.195 4.365 4.532 4.71 4.959 5.269 5.526 5.571] % Wolfspeed XML derived V  diode_TjVec=[-55 25 150 900 1000] % Wolfspeed XML derived degC  diode_VfVec=[.5, .7, .9, 1.3, 1.7, 2.1, 2.5] % Parameter not set V  diode_IfVec=[0 0.21 1.74 3.58 8.82 11.74 29.79 49.06 71.98 98.06 121.2 141.4 161.2 181.3 221.3 260.9 300 306.3] % Wolfspeed XML derived A  diode_IrMat=[1e-06, 2e-06, 5e-06, 1e-05, 2.5e-05, 5e-05, .0001; 2e-06, 5e-06, 1e-05, 4e-05, 8e-05, .0002, .0005] % Parameter not set A  diode_VrMat=[10, 100, 200, 250, 300, 325, 350; 10, 70, 160, 220, 270, 300, 320] % Parameter not set V  diode_VrVec=[10, 20, 40, 50, 70, 80, 100] % Parameter not set V  diode_IrVec=[1e-06, 2e-06, 5e-06, 1e-05, 2e-05, 5e-05, .0001] % Parameter not set A  diode_Vr=-600 % Parameter not set V  diode_Ls=150 % Parameter not set nH  diode_Erec=0.03 % Parameter not set J  diode_rec_loss_model=ee.enum.diode.reverseRecoveryModel.fixed  diode_ErecVal=0 % Parameter not set J  diode_scaleWithIandV=false  diode_ErecMat=[0 0;0 0] % Wolfspeed XML derived J  diodeErecMat3D=zeros(2, 3, 2) J  diode_TjrecVec=[25 35] % Wolfspeed XML derived degC  diode_IfrecVec=[0 10] % Wolfspeed XML derived A  diodeVrecVec=[0, 100] V  diode_IrecVal=10 % Parameter not set A  diode_VrecVal=10 % Wolfspeed XML derived V  diode_tFilter=1 / 1000 / 100 % Parameter not set s  separateThermalPortForDiode=false  thermal_network_parameterization=ee.enum.thermalNetworkTopology.external  Rth=[.03, .2] % Parameter not set K/W  Rth_Cauer=[0.01728 0.0646 0.05315 0.1045] % Wolfspeed XML derived K/W  Rth_Foster=[.08, .14, .22, .16] % Parameter not set K/W  thermal_mass_parameterization=ee.enum.thermalNetwork.thermalmass  thermal_mass=[3, 25] % Parameter not set J/K  thermal_mass_Cauer=[0.00466 0.0158 0.0642 0.264] % Wolfspeed XML derived J/K  thermal_mass_Foster=[.001, .005, .05, .5] % Parameter not set J/K  thermal_time_constant=[.1, 5] % Parameter not set s  thermal_time_constant_Cauer=[.1, 1, 5] % Parameter not set s  thermal_time_constant_Foster=[7e-05, .0007, .01, .08] % Parameter not set s  thermal_mass_initial_temperatures=[25, 25] % Parameter not set degC  thermal_mass_initial_temperatures_Cauer=[25 25 25 25] % Wolfspeed XML derived degC  junction_thermal_mass=0.01 % Parameter not set J/K  Tvec_initial_Foster=[25, 25, 25, 25] % Parameter not set degC  RthDiode=[.03, .2] % Parameter not set K/W  RthCauerDiode=[0.01728 0.0646 0.05315 0.1045] % Wolfspeed XML derived K/W  RthFosterDiode=[.03, .2] % Parameter not set K/W  thermalMassDiode=[3, 25] % Parameter not set J/K  thermalMassCauerDiode=[0.00466 0.0158 0.0642 0.264] % Wolfspeed XML derived J/K  thermalMassFosterDiode=[33, 50] % Parameter not set J/K  thermalTauDiode=[.1, 5] % Parameter not set s  thermalTauCauerDiode=[.1, 1, 5] % Parameter not set s  thermalTauFosterDiode=[1, 10] % Parameter not set s  thermalMassInitTempDiode=[25, 25] % Parameter not set degC  thermalMassInitTempCauerDiode=[25 25 25 25] % Wolfspeed XML derived degC  junctionthermalMassDiode=0.1 % Parameter not set J/K  TVecInitialFosterDiode=[25, 25, 25, 25] % Parameter not set degC  no_thermal_network=0 % Parameter not set  mosfet_junction_temperature_specify=on  mosfet_junction_temperature_priority=High  mosfet_junction_temperature=simTemp_K K  mosfet_junction_temperature_nominal_specify=off  mosfet_junction_temperature_nominal_value=1  mosfet_junction_temperature_nominal_unit=degC  diode_junction_temperature_specify=off  diode_junction_temperature_priority=None  diode_junction_temperature=simTemp_K K  diode_junction_temperature_nominal_specify=off  diode_junction_temperature_nominal_value=1  diode_junction_temperature_nominal_unit=degC  Qj_specify=off  Qj_priority=None  Qj=0 W  Qj_nominal_specify=off  Qj_nominal_value=1  Qj_nominal_unit=W  accumulatedSwitchingLosses_specify=off  accumulatedSwitchingLosses_priority=None  accumulatedSwitchingLosses=0 J
      settings: AttributesFormatString=Wolfspeed:C3M0010090K
  SL_PS : nesl_utility/Simulink-PS Converter  PhysicalDomain=network_engine_domain  SubClassName=ps_input  LeftPortType=input  RightPortType=output  PseudoPeriodic=off  Frequencies=[]  NoiseDistribution=none  NoiseParameters=[]  Unit=1  AffineConversion=off  FilteringAndDerivatives=provide  SimscapeFilterOrder=1  InputFilterTimeConstant=0.001  UdotUserProvided=0
  Temperature Source : fl_lib/Thermal/Thermal Sources/Temperature Source  temperature=simTemp_K K
  Thermal Resistor : ee_lib/Passive/Thermal/Thermal Resistor  R=1e-3 K/W  T_specify=off  T_priority=None  T=0 K  T_nominal_specify=off  T_nominal_value=1  T_nominal_unit=K  Q_specify=off  Q_priority=None  Q=0 W  Q_nominal_specify=off  Q_nominal_value=1  Q_nominal_unit=W
  D : PMIOPort  Side=Left
  S : PMIOPort  Port=2  Side=Right
  wires:
  G/1 -> SL_PS/1
  connections:
  SL_PS/RConn1 -- MOSFET/LConn1
  MOSFET/RConn1 -- D/RConn1
  MOSFET/RConn2 -- S/RConn1
  MOSFET/LConn2 -- Thermal Resistor/LConn1
  Thermal Resistor/RConn1 -- Temperature Source/LConn1

== system ConverterPlantLibrary/Non-Isolated DC-DC Converters/Non-Isolated DC-DC Converter/NonIsolatedDCDCVariant/SynchronousBuck/SyncSwitch/IdealSwitch ==
  G : Inport
  SL_PS : nesl_utility/Simulink-PS Converter  PhysicalDomain=network_engine_domain  SubClassName=ps_input  LeftPortType=input  RightPortType=output  PseudoPeriodic=off  Frequencies=[]  NoiseDistribution=none  NoiseParameters=[]  Unit=1  AffineConversion=off  FilteringAndDerivatives=provide  SimscapeFilterOrder=1  InputFilterTimeConstant=0.001  UdotUserProvided=0
  Switch : ee_lib/Semiconductors & Converters/Ideal Semiconductor Switch  port_option=ee.enum.controlport.ps  Ron=RdsOn_SI Ohm  Goff=GdsOff_SI 1/Ohm  Vth=Vth_SI V  diode_param=ee.enum.semiconductors.protectionDiode.nodynamics  diode_Vf=VfBody_SI V  diode_Ron=RdBody_SI Ohm  diode_Goff=GdBody_SI 1/Ohm  diode_C=50e-9 F  diode_iRM=-235 A  diode_iF=300 A  diode_idot=-50 A/us  diode_trr_param=ee.enum.converters.diodetrr.trr_factor  diode_trr_factor=3  diode_trr=15 us  diode_Qrr=1500 s*uA
  D : PMIOPort  Side=Left
  S : PMIOPort  Port=2  Side=Right
  wires:
  G/1 -> SL_PS/1
  connections:
  SL_PS/RConn1 -- Switch/LConn1
  Switch/RConn1 -- D/RConn1
  Switch/RConn2 -- S/RConn1

== system ConverterPlantLibrary/Non-Isolated DC-DC Converters/Non-Isolated DC-DC Converter/NonIsolatedDCDCVariant/SynchronousBuck/SyncSwitch/SwitchingMOSFETwithThermal ==
  G : Inport
  MOSFET : ee_lib/Semiconductors & Converters/MOSFET (Ideal, Switching)  PartSpecification="{\"CollectionId\":\"SimscapeElectrical\",\"CollectionVersion\":\"1.0.0\",\"DatasetId\":\"Wolfspeed|C3M0010090K|\",\"DisplayName\":\"Wolfspeed:C3M0010090K\"}"  port_option=ee.enum.controlport.ps  Rds=0.03 % Datasheet derived Ohm  Goff=1e-05 S  Vth=2.41 % Wolfspeed XML derived V  diode_param=ee.enum.semiconductors.protectionDiode.nodynamics  diode_Vf=0.8 V  diode_Ron=1e-3 Ohm  diode_Goff=1e-5 S  diode_C=50e-9 % Parameter not set F  diode_iRM=-235 % Parameter not set A  diode_iF=300 % Parameter not set A  diode_idot=-50 % Parameter not set A/us  diode_trr_param=ee.enum.converters.diodeReverseParam.trr_factor  diode_trr_factor=3 % Parameter not set  diode_trr=15 % Parameter not set us  diode_Qrr=1500 % Parameter not set s*uA  ids_specify=off  ids_priority=None  ids=0 A  ids_nominal_specify=off  ids_nominal_value=1  ids_nominal_unit=A  vds_specify=off  vds_priority=None  vds=0 V  vds_nominal_specify=off  vds_nominal_value=1  vds_nominal_unit=V  vgs_specify=off  vgs_priority=None  vgs=0 V  vgs_nominal_specify=off  vgs_nominal_value=1  vgs_nominal_unit=V  thermal_loss_option=ee.enum.converters.thermalLossOption.tabulated2d  Von_data=[-2.582 -2.511 -2.366 -2.145 -1.916 -1.601 -1.356 -1.103 -0.7517 -0.4733 -0.3149 -0.1528 -0.0851 -0.05 0 0.094 0.161 0.305 0.51 0.83 1.31 1.61 1.908 2.42 2.766 3.142 3.373 3.713;-2.869 -2.757 -2.58 -2.311 -2.042 -1.683 -1.41 -1.134 -0.7615 -0.4747 -0.3153 -0.149 -0.0819 -0.0469 0 0.09975 0.154 0.303 0.509 0.819 1.241 1.581 1.9 2.39 2.758 3.144 3.4 3.78;-4.55 -4.355 -4.055 -3.569 -3.136 -2.526 -2.113 -1.659 -1.117 -0.7115 -0.4389 -0.2087 -0.116 -0.0674 0 0.123 0.239 0.421 0.701 1.175 1.743 2.252 2.7 3.4 4 4.52 5.03 5.4;-5.005 -4.791 -4.461 -3.926 -3.45 -2.779 -2.324 -1.825 -1.229 -0.7826 -0.4828 -0.2296 -0.1276 -0.07414 0 0.1353 0.2629 0.4631 0.7711 1.292 1.917 2.477 2.97 3.74 4.4 4.972 5.533 5.94] % Wolfspeed XML derived V  Tj=[-55 25 150 900] % Wolfspeed XML derived degC  Iout_data=[-311.6 -300 -280 -250 -220 -180 -150 -120 -80 -50 -32.71 -15.83 -9 -5.52 0 9 15.6 30 50 80 120 150 180 220 250 280 300 327] % Wolfspeed XML derived A  tabulateWithVds=true  Eon_data=[0 0.00054 0.00072 0.0009 0.00109 0.00126 0.00142 0.00163 0.0018;0 0.00036 0.00048 0.0006 0.00073 0.00084 0.00095 0.00109 0.0012;0 0.00037 0.00049 0.00061 0.00074 0.00085 0.00097 0.00111 0.00122;0 0.00041 0.00054 0.00067 0.00081 0.00094 0.00106 0.00122 0.00135;0 0.00041 0.00054 0.00067 0.00081 0.00094 0.00106 0.00122 0.00135] % Wolfspeed XML derived J  Eoff_data=[0 0.00013 0.0002 0.00022 0.00026 0.00033 0.00044 0.00055 0.00067;0 0.00014 0.00021 0.00024 0.00028 0.00036 0.00047 0.00059 0.00072;0 0.00016 0.00024 0.00027 0.00031 0.00041 0.00054 0.00067 0.00082;0 0.00016 0.00024 0.00027 0.00032 0.00041 0.00054 0.00068 0.00083;0 0.00016 0.00024 0.00027 0.00032 0.00041 0.00054 0.00068 0.00083] % Wolfspeed XML derived J  Eon_data_3D=reshape([0;0;0;0;0;0;0;0;0;0;0;0;0;0;0;0;0;0;0;0;0;0;0;0;0;0;0;0;0;0;0;0;0;0;0;0;0;0;0;0;0;0;0;0;0;0;0;0;0;0;0;0;0;0;0;0;0;0;0;0;0;0;0;0;0;0;0;0;0;0;0;0;0;0;0;0;0;0;0;0;0;0;0;0;0;0;0;0;0;0;0;0;0;0;0;0.00025;0.00017;0.00017;0.00019;0.00019;0.00035;0.00024;0.00024;0.00026;0.00026;0.00044;0.00029;0.0003;0.00033;0.00033;0.00051;0.00034;0.00035;0.00038;0.00038;0.0006;0.0004;0.00041;0.00045;0.00045;0.00072;0.00048;0.00049;0.00054;0.00054;0.00079;0.00053;0.00054;0.00059;0.00059;0.00087;0.00058;0.00059;0.00065;0.00065;0;0;0;0;0;0.00054;0.00036;0.00037;0.00041;0.00041;0.00072;0.00048;0.00049;0.00054;0.00054;0.0009;0.0006;0.00061;0.00067;0.00067;0.00109;0.00073;0.00074;0.00081;0.00081;0.00126;0.00084;0.00085;0.00094;0.00094;0.00142;0.00095;0.00097;0.00106;0.00106;0.00163;0.00109;0.00111;0.00122;0.00122;0.0018;0.0012;0.00122;0.00135;0.00135],[5 9 4]) % Wolfspeed XML derived J  Eoff_data_3D=reshape([0;0;0;0;0;0;0;0;0;0;0;0;0;0;0;0;0;0;0;0;0;0;0;0;0;0;0;0;0;0;0;0;0;0;0;0;0;0;0;0;0;0;0;0;0;0;0;0;0;0;0;0;0;0;0;0;0;0;0;0;0;0;0;0;0;0;0;0;0;0;0;0;0;0;0;0;0;0;0;0;0;0;0;0;0;0;0;0;0;0;0;0;0;0;0;8e-05;8e-05;0.0001;0.0001;0.0001;0.00014;0.00015;0.00017;0.00017;0.00017;0.00016;0.00018;0.0002;0.0002;0.0002;0.00017;0.00018;0.00021;0.00021;0.00021;0.00023;0.00025;0.00029;0.00029;0.00029;0.0003;0.00032;0.00037;0.00037;0.00037;0.00038;0.00041;0.00046;0.00047;0.00047;0.00046;0.00049;0.00056;0.00057;0.00057;0;0;0;0;0;0.00013;0.00014;0.00016;0.00016;0.00016;0.0002;0.00021;0.00024;0.00024;0.00024;0.00022;0.00024;0.00027;0.00027;0.00027;0.00026;0.00028;0.00031;0.00032;0.00032;0.00033;0.00036;0.00041;0.00041;0.00041;0.00044;0.00047;0.00054;0.00054;0.00054;0.00055;0.00059;0.00067;0.00068;0.00068;0.00067;0.00072;0.00082;0.00083;0.00083],[5 9 4]) % Wolfspeed XML derived J  Tj_loss=[-55 25 150 900 1000] % Wolfspeed XML derived degC  Iout_data_loss=[0 12.2 26.4 38.8 52.6 66 78.9 91 103.3] % Wolfspeed XML derived A  Vds_loss=[-100 0 400 600] % Wolfspeed XML derived V  Eon_scalar=22.86e-3 % Parameter not set J  Eoff_scalar=17.14e-3 % Parameter not set J  Voff=300 % Parameter not set V  Iout_scalar=600 % Parameter not set A  useCurrentFromPreviousCycle=false % Parameter not set  useVoltageFromPreviousCycle=false % Parameter not set  diodeModelType=ee.enum.converters.diodeModelType.pwl  diodeTableType=ee.enum.diode.tableType.VfMat  diode_ReverseIVType=ee.enum.diode.diodeReverseIV.constant  diode_IfMat=[.07, .12, .19, 1.75, 4.24, 7.32, 11.2; .16, .3, .72, 2.14, 4.02, 6.35, 9.12] % Parameter not set A  diode_VfMat=[0 0.718 3.358 3.487 3.935 4.083 4.682 5.031 5.458 5.658 5.958 6.147 6.32 6.575 6.799 7.03 7.267 7.29;0 0.718 2.914 3.116 3.391 3.497 3.954 4.289 4.612 4.933 5.187 5.39 5.581 5.763 6.107 6.422 6.711 6.76;0 0.718 2.4 2.6 2.8 2.982 3.45 3.789 4.099 4.428 4.661 4.85 5.035 5.233 5.51 5.855 6.14 6.19;0 0.6462 2.16 2.34 2.52 2.684 3.105 3.41 3.689 3.985 4.195 4.365 4.532 4.71 4.959 5.269 5.526 5.571;0 0.6462 2.16 2.34 2.52 2.684 3.105 3.41 3.689 3.985 4.195 4.365 4.532 4.71 4.959 5.269 5.526 5.571] % Wolfspeed XML derived V  diode_TjVec=[-55 25 150 900 1000] % Wolfspeed XML derived degC  diode_VfVec=[.5, .7, .9, 1.3, 1.7, 2.1, 2.5] % Parameter not set V  diode_IfVec=[0 0.21 1.74 3.58 8.82 11.74 29.79 49.06 71.98 98.06 121.2 141.4 161.2 181.3 221.3 260.9 300 306.3] % Wolfspeed XML derived A  diode_IrMat=[1e-06, 2e-06, 5e-06, 1e-05, 2.5e-05, 5e-05, .0001; 2e-06, 5e-06, 1e-05, 4e-05, 8e-05, .0002, .0005] % Parameter not set A  diode_VrMat=[10, 100, 200, 250, 300, 325, 350; 10, 70, 160, 220, 270, 300, 320] % Parameter not set V  diode_VrVec=[10, 20, 40, 50, 70, 80, 100] % Parameter not set V  diode_IrVec=[1e-06, 2e-06, 5e-06, 1e-05, 2e-05, 5e-05, .0001] % Parameter not set A  diode_Vr=-600 % Parameter not set V  diode_Ls=150 % Parameter not set nH  diode_Erec=0.03 % Parameter not set J  diode_rec_loss_model=ee.enum.diode.reverseRecoveryModel.fixed  diode_ErecVal=0 % Parameter not set J  diode_scaleWithIandV=false  diode_ErecMat=[0 0;0 0] % Wolfspeed XML derived J  diodeErecMat3D=zeros(2, 3, 2) J  diode_TjrecVec=[25 35] % Wolfspeed XML derived degC  diode_IfrecVec=[0 10] % Wolfspeed XML derived A  diodeVrecVec=[0, 100] V  diode_IrecVal=10 % Parameter not set A  diode_VrecVal=10 % Wolfspeed XML derived V  diode_tFilter=1 / 1000 / 100 % Parameter not set s  separateThermalPortForDiode=false  thermal_network_parameterization=ee.enum.thermalNetworkTopology.external  Rth=[.03, .2] % Parameter not set K/W  Rth_Cauer=[0.01728 0.0646 0.05315 0.1045] % Wolfspeed XML derived K/W  Rth_Foster=[.08, .14, .22, .16] % Parameter not set K/W  thermal_mass_parameterization=ee.enum.thermalNetwork.thermalmass  thermal_mass=[3, 25] % Parameter not set J/K  thermal_mass_Cauer=[0.00466 0.0158 0.0642 0.264] % Wolfspeed XML derived J/K  thermal_mass_Foster=[.001, .005, .05, .5] % Parameter not set J/K  thermal_time_constant=[.1, 5] % Parameter not set s  thermal_time_constant_Cauer=[.1, 1, 5] % Parameter not set s  thermal_time_constant_Foster=[7e-05, .0007, .01, .08] % Parameter not set s  thermal_mass_initial_temperatures=[25, 25] % Parameter not set degC  thermal_mass_initial_temperatures_Cauer=[25 25 25 25] % Wolfspeed XML derived degC  junction_thermal_mass=0.01 % Parameter not set J/K  Tvec_initial_Foster=[25, 25, 25, 25] % Parameter not set degC  RthDiode=[.03, .2] % Parameter not set K/W  RthCauerDiode=[0.01728 0.0646 0.05315 0.1045] % Wolfspeed XML derived K/W  RthFosterDiode=[.03, .2] % Parameter not set K/W  thermalMassDiode=[3, 25] % Parameter not set J/K  thermalMassCauerDiode=[0.00466 0.0158 0.0642 0.264] % Wolfspeed XML derived J/K  thermalMassFosterDiode=[33, 50] % Parameter not set J/K  thermalTauDiode=[.1, 5] % Parameter not set s  thermalTauCauerDiode=[.1, 1, 5] % Parameter not set s  thermalTauFosterDiode=[1, 10] % Parameter not set s  thermalMassInitTempDiode=[25, 25] % Parameter not set degC  thermalMassInitTempCauerDiode=[25 25 25 25] % Wolfspeed XML derived degC  junctionthermalMassDiode=0.1 % Parameter not set J/K  TVecInitialFosterDiode=[25, 25, 25, 25] % Parameter not set degC  no_thermal_network=0 % Parameter not set  mosfet_junction_temperature_specify=on  mosfet_junction_temperature_priority=High  mosfet_junction_temperature=simTemp_K K  mosfet_junction_temperature_nominal_specify=off  mosfet_junction_temperature_nominal_value=1  mosfet_junction_temperature_nominal_unit=degC  diode_junction_temperature_specify=off  diode_junction_temperature_priority=None  diode_junction_temperature=simTemp_K K  diode_junction_temperature_nominal_specify=off  diode_junction_temperature_nominal_value=1  diode_junction_temperature_nominal_unit=degC  Qj_specify=off  Qj_priority=None  Qj=0 W  Qj_nominal_specify=off  Qj_nominal_value=1  Qj_nominal_unit=W  accumulatedSwitchingLosses_specify=off  accumulatedSwitchingLosses_priority=None  accumulatedSwitchingLosses=0 J
      settings: AttributesFormatString=Wolfspeed:C3M0010090K
  SL_PS : nesl_utility/Simulink-PS Converter  PhysicalDomain=network_engine_domain  SubClassName=ps_input  LeftPortType=input  RightPortType=output  PseudoPeriodic=off  Frequencies=[]  NoiseDistribution=none  NoiseParameters=[]  Unit=1  AffineConversion=off  FilteringAndDerivatives=provide  SimscapeFilterOrder=1  InputFilterTimeConstant=0.001  UdotUserProvided=0
  Temperature Source : fl_lib/Thermal/Thermal Sources/Temperature Source  temperature=simTemp_K K
  Thermal Resistor : ee_lib/Passive/Thermal/Thermal Resistor  R=1e-3 K/W  T_specify=off  T_priority=None  T=0 K  T_nominal_specify=off  T_nominal_value=1  T_nominal_unit=K  Q_specify=off  Q_priority=None  Q=0 W  Q_nominal_specify=off  Q_nominal_value=1  Q_nominal_unit=W
  D : PMIOPort  Side=Left
  S : PMIOPort  Port=2  Side=Right
  wires:
  G/1 -> SL_PS/1
  connections:
  SL_PS/RConn1 -- MOSFET/LConn1
  MOSFET/RConn1 -- D/RConn1
  MOSFET/RConn2 -- S/RConn1
  MOSFET/LConn2 -- Thermal Resistor/LConn1
  Thermal Resistor/RConn1 -- Temperature Source/LConn1

== system ConverterPlantLibrary/Non-Isolated DC-DC Converters/Non-Isolated DC-DC Converter/NonIsolatedDCDCVariant/SynchronousBuckBoost/MainSwitch/IdealSwitch ==
  G : Inport
  SL_PS : nesl_utility/Simulink-PS Converter  PhysicalDomain=network_engine_domain  SubClassName=ps_input  LeftPortType=input  RightPortType=output  PseudoPeriodic=off  Frequencies=[]  NoiseDistribution=none  NoiseParameters=[]  Unit=1  AffineConversion=off  FilteringAndDerivatives=provide  SimscapeFilterOrder=1  InputFilterTimeConstant=0.001  UdotUserProvided=0
  Switch : ee_lib/Semiconductors & Converters/Ideal Semiconductor Switch  port_option=ee.enum.controlport.ps  Ron=RdsOn_SI Ohm  Goff=GdsOff_SI 1/Ohm  Vth=Vth_SI V  diode_param=ee.enum.semiconductors.protectionDiode.nodynamics  diode_Vf=VfBody_SI V  diode_Ron=RdBody_SI Ohm  diode_Goff=GdBody_SI 1/Ohm  diode_C=50e-9 F  diode_iRM=-235 A  diode_iF=300 A  diode_idot=-50 A/us  diode_trr_param=ee.enum.converters.diodetrr.trr_factor  diode_trr_factor=3  diode_trr=15 us  diode_Qrr=1500 s*uA
  D : PMIOPort  Side=Left
  S : PMIOPort  Port=2  Side=Right
  wires:
  G/1 -> SL_PS/1
  connections:
  Switch/RConn2 -- S/RConn1
  Switch/RConn1 -- D/RConn1
  SL_PS/RConn1 -- Switch/LConn1
